simulink model "gtm_design"  (R2021b)
settings: Solver=ode15s  StartTime=0.0  StopTime=15  FixedStep=0.005  MaxStep=0.005  MinStep=0.0025
StopFcn:
  | MWSout=grabmws(bdroot);
  | MWSout.lastrun=datestr(now);
values from neighbouring files (symbols this model uses):
  s = tf('s')    [SingleDOF.m]    (also in main.m; newmain.m)
undefined symbols (not defined in the file or in its folder): Aero, aftfuel, aftfuel_pos, AILL, AILLC, AILR, AILRC, alpha_deg, altitude_ft, Ax_g, Ay_g, Az_g, b, beta_deg, bias, BRAKEC, Cbar, cg_pos0, cg_shift_gear, DamageCase, DamageModels, DamageOnsetTime, Earth, ELLIB, ELLIBC, ELLOB, ELLOBC, ELRIB, ELRIBC, ELROB, ELROBC, engl_ang, engl_pos, engr_ang, engr_pos, FLAPLIB, FLAPLIC, FLAPLOB, FLAPLOC, FLAPRIB, FLAPRIC, FLAPROB, FLAPROC, ft, FuelUsed_Init, fwdfuel, fwdfuel_pos, GEAR, GEARC, Inertia0, Inertia_shift_gear, Ixx_model, Iyy_model, Izz_model, KTAS, LandingGear, LengON, LinearizeModeOn, NAV_altitude_m, NAV_latitude_deg ... (+51)
libraries: simulink_extras x64, simulink_need_slupdate x30, LPVBlockLibrary x23, aerolibconvert2 x6, aerolibtransform2 x5, uavalgslib x4, UserContent_lib x3, simulink x3, robotcorelib x1, uavutilslib x1
(part 2 of 8)

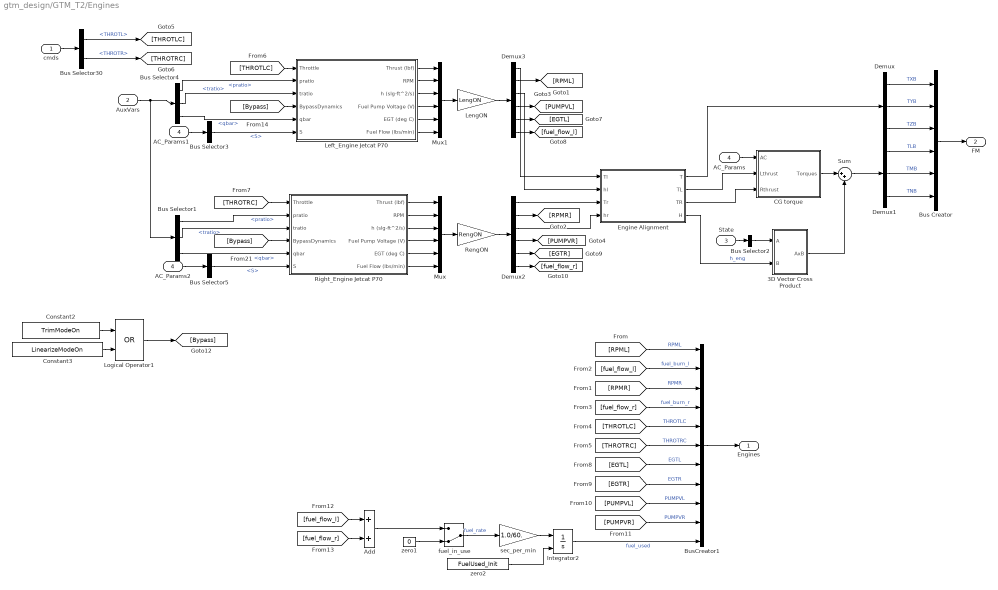
== system gtm_design/GTM_T2/Engines ==
  cmds : Inport
  AuxVars : Inport  Port=2
  State : Inport  Port=3
  AC_Params : Inport  Port=4
  3D Vector Cross Product : Subsystem
  AC_Params1 : InportShadow  Port=4
  AC_Params2 : InportShadow  Port=4
  Add : Sum
  Bus Creator : BusCreator  Inputs=6
  Bus Selector1 : BusSelector  OutputSignals=pratio,tratio,qbar
  Bus Selector2 : BusSelector  OutputSignals=pb,qb,rb  OutputAsBus=on
  Bus Selector3 : BusSelector  OutputSignals=S
  Bus Selector30 : BusSelector  OutputSignals=THROTL,THROTR
  Bus Selector4 : BusSelector  OutputSignals=pratio,tratio,qbar
  Bus Selector5 : BusSelector  OutputSignals=S
  BusCreator1 : BusCreator  Inputs=11
  CG torque : Subsystem
  Constant2 : Constant  Value=TrimModeOn
  Constant3 : Constant  Value=LinearizeModeOn
  Demux : Demux  Outputs=3
  Demux1 : Demux  Outputs=3
  Demux2 : Demux  Outputs=6
  Demux3 : Demux  Outputs=6
  Engine Alignment : MATLAB Function  TreatAsAtomicUnit=on
  Integrator2 : Integrator  InitialConditionSource=external
  Left_Engine Jetcat P70 : Subsystem
      mask init:
      | % Curve fit parameters for Jetcat P70 Model
      | % Coeff_thrust   = [0.000028864242464  -0.001914835880159 0.105916926095459  -1.251646340183624 ];
      | Coeff_thrust   = [0.000014847593013,  0, 0, 0.412662356277121];
      | Coeff_throttle = [0.000033035538475  -0.008354385314499 1.191126728328792 31.518959847101669];
      | Coeff_fuelflow = [0.000046800927870  -0.000779344124807 0.122178501497750];
      | Coeff_tau      = [ -2.2400e-02   2.9948e+00];
      | Coeff_EGT      = [ 2E-5, -0.0036,0.2342,-8.0496,664.99]; %EGT model, deg C
      | Coeff_dynamics = [ -.074 7.1];
      | fuelpump_table = [0 0.576	0.625	0.6985	0.7845	0.8575	0.919	0.9805	1.0415	1.1025...
      |                     1.1515	1.262	1.287	1.373	1.52	1.618	1.74	1.887	1.973...
      |                     2.12	2.255	2.4385	2.647	2.7575	2.9905	3.162]; %volts, table of fuel pump voltages
      | fuelflow_table = [0,0.0794,0.0876,0.102,0.1149,0.1275,0.1379,0.1487,0.1586,0.1671,...
      |                     0.1775,0.1858,0.194,0.2038,0.2206,0.2405,0.2566,0.2746,0.2921,0.3102,...
      |                     0.3266,0.3445,0.3533,0.3611,0.3866,0.4083;]*2; %lbs/min,   FULL fuel flow rates corresponding to pump voltages (fuelpump_table)  
      | % Equvalent Shaft parameters for engine
      | shaft_dia = 0.75/12.0;       % diameter of rotating turbine in feet 
      | shaft_len = 6.25/12.0;       % length of rotating turbine in feet   
      | density   = 15.2;            % mass density of steel in slugs/ft^3 
      | 
      | 
      | A = [-1.336,-0.7314;1,0;];
      | B = [1;0];
      | C = [-0.1474   0.7314];
      | D = 0;
  LengON : Gain  Gain=LengON  SaturateOnIntegerOverflow=on  OutDataTypeStr=Inherit: Same as input  ParamDataTypeStr=Inherit: Same as input
  Logical Operator1 : Logic  Operator=OR  AllPortsSameDT=off  OutDataTypeStr=boolean
  Mux : Mux  Inputs=6
  Mux1 : Mux  Inputs=6
  RengON : Gain  Gain=RengON  SaturateOnIntegerOverflow=on  OutDataTypeStr=Inherit: Same as input  ParamDataTypeStr=Inherit: Same as input
  Right_Engine Jetcat P70 : Subsystem
      mask init: same as gtm_design/GTM_T2/Engines/Left_Engine Jetcat P70
  Sum : Sum  Inputs=|++
  fuel_in_use : ManualSwitch  CurrentSetting=0
  sec_per_min : Gain  Gain=1.0/60.  SaturateOnIntegerOverflow=on  OutDataTypeStr=Inherit: Same as input  ParamDataTypeStr=Inherit: Same as input
  zero1 : Constant  Value=0
  zero2 : Constant  Value=FuelUsed_Init
  Engines : Outport
  FM : Outport  Port=2  PortDimensions=6
  wires:
  cmds/1 -> Bus Selector30/1
  Demux/2 -> Bus Creator/2  "TYB"
  State/1 -> Bus Selector2/1
  Bus Selector2/1 -> 3D Vector Cross Product/1(A)
  Demux/3 -> Bus Creator/3  "TZB"
  AuxVars/1 -> Bus Selector1/1, Bus Selector4/1
  AC_Params/1 -> CG torque/1(AC)
  Bus Creator/1 -> FM/1
  Bus Selector30/1 -> [THROTLC]  "<THROTL>"
  Bus Selector30/2 -> [THROTRC]  "<THROTR>"
  [THROTRC] -> BusCreator1/6  "THROTRC"
  [THROTLC] -> BusCreator1/5  "THROTLC"
  [fuel_flow_r] -> BusCreator1/4  "fuel_burn_r"
  [fuel_flow_l] -> BusCreator1/2  "fuel_burn_l"
  [RPMR] -> BusCreator1/3  "RPMR"
  [RPML] -> BusCreator1/1  "RPML"
  BusCreator1/1 -> Engines/1
  [EGTL] -> BusCreator1/7  "EGTL"
  [EGTR] -> BusCreator1/8  "EGTR"
  [PUMPVL] -> BusCreator1/9  "PUMPVL"
  [PUMPVR] -> BusCreator1/10  "PUMPVR"
  sec_per_min/1 -> Integrator2/1
  fuel_in_use/1 -> sec_per_min/1  "fuel_rate"
  Integrator2/1 -> BusCreator1/11  "fuel_used"
  zero2/1 -> Integrator2/2
  [fuel_flow_l] -> Add/1
  [fuel_flow_r] -> Add/2
  zero1/1 -> fuel_in_use/2
  Add/1 -> fuel_in_use/1
  Demux/1 -> Bus Creator/1  "TXB"
  Engine Alignment/4(H) -> 3D Vector Cross Product/2(B)  "h_eng"
  Engine Alignment/1(T) -> Demux/1
  Engine Alignment/2(TL) -> CG torque/2(Lthrust)
  Engine Alignment/3(TR) -> CG torque/3(Rthrust)
  CG torque/1(Torques) -> Sum/1
  3D Vector Cross Product/1(AxB) -> Sum/2
  Sum/1 -> Demux1/1
  Demux1/1 -> Bus Creator/4  "TLB"
  Demux1/2 -> Bus Creator/5  "TMB"
  Demux1/3 -> Bus Creator/6  "TNB"
  Mux/1 -> RengON/1
  RengON/1 -> Demux2/1
  Demux2/1 -> Engine Alignment/3(Tr)
  Demux2/2 -> [RPMR]
  Demux2/3 -> Engine Alignment/4(hr)
  Demux2/4 -> [PUMPVR]
  Demux2/5 -> [EGTR]
  Demux2/6 -> [fuel_flow_r]
  Mux1/1 -> LengON/1
  LengON/1 -> Demux3/1
  Demux3/1 -> Engine Alignment/1(Tl)
  Demux3/2 -> [RPML]
  Demux3/3 -> Engine Alignment/2(hl)
  Demux3/4 -> [PUMPVL]
  Demux3/5 -> [EGTL]
  Demux3/6 -> [fuel_flow_l]
  Constant3/1 -> Logical Operator1/2
  Constant2/1 -> Logical Operator1/1
  Logical Operator1/1 -> [Bypass]
  Left_Engine Jetcat P70/1(Thrust (lbf)) -> Mux1/1
  Left_Engine Jetcat P70/2(RPM) -> Mux1/2
  Left_Engine Jetcat P70/3(h (slg-ft^2/s)) -> Mux1/3
  Left_Engine Jetcat P70/4(Fuel Pump Voltage (V)) -> Mux1/4
  Left_Engine Jetcat P70/5(EGT (deg C)) -> Mux1/5
  Left_Engine Jetcat P70/6(Fuel Flow (lbs/min)) -> Mux1/6
  Right_Engine Jetcat P70/1(Thrust (lbf)) -> Mux/1
  Right_Engine Jetcat P70/2(RPM) -> Mux/2
  Right_Engine Jetcat P70/3(h (slg-ft^2/s)) -> Mux/3
  Right_Engine Jetcat P70/4(Fuel Pump Voltage (V)) -> Mux/4
  Right_Engine Jetcat P70/5(EGT (deg C)) -> Mux/5
  Right_Engine Jetcat P70/6(Fuel Flow (lbs/min)) -> Mux/6
  AC_Params2/1 -> Bus Selector5/1
  AC_Params1/1 -> Bus Selector3/1
  [THROTRC] -> Right_Engine Jetcat P70/1(Throttle)
  [THROTLC] -> Left_Engine Jetcat P70/1(Throttle)
  Bus Selector4/1 -> Left_Engine Jetcat P70/2(pratio)  "<pratio>"
  Bus Selector4/2 -> Left_Engine Jetcat P70/3(tratio)  "<tratio>"
  [Bypass] -> Left_Engine Jetcat P70/4(BypassDynamics)
  Bus Selector4/3 -> Left_Engine Jetcat P70/5(qbar)  "<qbar>"
  Bus Selector3/1 -> Left_Engine Jetcat P70/6(S)  "<S>"
  Bus Selector1/1 -> Right_Engine Jetcat P70/2(pratio)  "<pratio>"
  Bus Selector1/2 -> Right_Engine Jetcat P70/3(tratio)  "<tratio>"
  [Bypass] -> Right_Engine Jetcat P70/4(BypassDynamics)
  Bus Selector1/3 -> Right_Engine Jetcat P70/5(qbar)  "<qbar>"
  Bus Selector5/1 -> Right_Engine Jetcat P70/6(S)  "<S>"

== system gtm_design/GTM_T2/Gravity ==
  AuxVars : Inport
  Params : Inport  Port=2
  Bus Selector1 : BusSelector  OutputSignals=DCM
  Bus Selector6 : BusSelector  OutputSignals=mass
  Ground : Ground
  Ground1 : Ground
  Mux : Mux  Inputs=[3 3]
  Mux1 : Mux  Inputs=3
  Product : Product  Multiplication=Matrix(*)  RndMeth=Zero
  Product1 : Product  RndMeth=Zero
  acc due to gravity (ft/s^2) : Constant  Value=32.17405
  FM : Outport
  wires:
  acc due to gravity (ft/s^2)/1 -> Product1/2
  Ground1/1 -> Mux/2
  Product1/1 -> Mux1/3
  Ground/1 -> Mux1/2, Mux1/1
  Mux1/1 -> Product/2
  Mux/1 -> FM/1
  Product/1 -> Mux/1
  Params/1 -> Bus Selector6/1
  AuxVars/1 -> Bus Selector1/1
  Bus Selector1/1 -> Product/1  "<DCM>"
  Bus Selector6/1 -> Product1/1  "<mass>"

== system gtm_design/GTM_T2/Landing Gear ==
  State : Inport
  Surfaces : Inport  Port=2
  ACParams : Inport  Port=3
  Bus Selector : BusSelector  OutputSignals=BRAKE,STEER,GEAR
  Bus Selector1 : BusSelector  OutputSignals=pb,qb,rb  OutputAsBus=on
  Bus Selector2 : BusSelector  OutputSignals=ub,vb,wb  OutputAsBus=on
  Bus Selector3 : BusSelector  OutputSignals=psi
  Bus Selector4 : BusSelector  OutputSignals=altitude
  Bus Selector5 : BusSelector  OutputSignals=phi,theta,psi  OutputAsBus=on
  Bus Selector6 : BusSelector  OutputSignals=CG  OutputAsBus=on
  Bus to Vector : BusToVector
  Bus to Vector1 : BusToVector
  Bus to Vector2 : BusToVector
  Gain : Gain  Gain=1/100
  LandingGear : Subsystem  mask{NoseWheelPos=LandingGear.NoseWheelPos, LeftMainPos=LandingGear.LeftMainPos, RightMainPos=LandingGear.RightMainPos, SpringConst=LandingGear.SpringConst, DampingConst=LandingGear.DampingConst, StrokeLength=LandingGear.StrokeLength, MountStiffness=LandingGear.MountStiff, MountDamping=LandingGear.MountDamping, RunwayAlt=runway_alt}
      mask prompts: NoseWheelPos "Nose Wheel Position [X,Y,Z]"; LeftMainPos "Left Main Position [X,Y,Z]"; RightMainPos "Right Main Position [X,Y,Z]"; SpringConst "Spring Constant [Nose,Left,Right]"; DampingConst "Damping Constant [Nose,Left,Right]"; StrokeLength "Stroke Length [Nose,Left,Right]"; MountStiffness "Mount Stiffness [Nose,Left,Right]"; MountDamping "Mount Damping [Nose,Left, Right]"; RunwayAlt "Runway Altitude"
      mask help:
      | Implements ground reaction force (if geardown is nonzero) for 3-wheel landing gear. Linear stiffness and damping are applied within stroke range, and (generally larger) mount stiffness and damping are applied beyond this range.
      |
      | Underlying gear.c function is from HL-20/LaRCsim, e.b.jackson@nasa.gov
  Mux : Mux  Inputs=2
  FM : Outport
  GearState : Outport  Port=2
  wires:
  Mux/1 -> FM/1
  Gain/1 -> LandingGear/7(Brake (0-1))
  LandingGear/3(Contact) -> GearState/1
  LandingGear/2(M_gear) -> Mux/2
  LandingGear/1(F_gear) -> Mux/1
  Bus Selector/3 -> LandingGear/9(geardown (0/1))  "<GEAR>"
  Bus Selector/2 -> LandingGear/8(Steer (deg))  "<STEER>"
  Bus Selector/1 -> Gain/1  "<BRAKE>"
  Bus Selector3/1 -> LandingGear/6(Heading (Rad))  "<psi>"
  Bus to Vector/1 -> LandingGear/4(pqr (Rad/sec))
  Bus Selector4/1 -> LandingGear/3(Altitude (ft))  "<altitude>"
  Bus to Vector2/1 -> LandingGear/2(EulerAngles (Rad))
  Bus Selector6/1 -> LandingGear/1(cg)
  Surfaces/1 -> Bus Selector/1
  State/1 -> Bus Selector1/1, Bus Selector2/1, Bus Selector3/1, Bus Selector4/1, Bus Selector5/1
  Bus Selector1/1 -> Bus to Vector/1
  Bus to Vector1/1 -> LandingGear/5(Vbody (ft/sec))
  Bus Selector2/1 -> Bus to Vector1/1
  Bus Selector5/1 -> Bus to Vector2/1
  ACParams/1 -> Bus Selector6/1

== system gtm_design/GTM_T2/Sensors ==
  EOM_State : Inport
  EOM_Xdot : Inport  Port=2
  AC_Params : Inport  Port=3
  AuxVars : Inport  Port=4
  SurfacePos : Inport  Port=5
  Engines : Inport  Port=6
  Air Data : Subsystem
  AuxVars1 : InportShadow  Port=4
  Bus Creator : BusCreator  Inputs=5
  Engine ECU 8 Hz : Subsystem  SystemSampleTime=round(1/Timestep/8)*Timestep
  MAG3 IMU : Subsystem
  MIDG II 50 Hz : Subsystem  SystemSampleTime=round(1/Timestep/50)*Timestep
  Surface Pots : Subsystem
  Terminator : Terminator
  Terminator1 : Terminator
  Sensors : Outport
  wires:
  AC_Params/1 -> Terminator1/1
  EOM_Xdot/1 -> Terminator/1
  Bus Creator/1 -> Sensors/1
  Air Data/1(AirData) -> Bus Creator/1  "AirData"
  MIDG II 50 Hz/1(MIDG) -> Bus Creator/2  "MIDG"
  Surface Pots/1(Pots) -> Bus Creator/4  "SurfacePos"
  Engine ECU 8 Hz/1(ECU) -> Bus Creator/5  "Engines"
  MAG3 IMU/1(MAG3) -> Bus Creator/3  "MAG3"
  Engines/1 -> Engine ECU 8 Hz/1(Engines)
  SurfacePos/1 -> Surface Pots/1(SurfacePos)
  AuxVars/1 -> Air Data/2(AuxVars), MIDG II 50 Hz/1(AuxVars)
  EOM_State/1 -> MIDG II 50 Hz/2(EOM_State), Air Data/1(EOM_State), MAG3 IMU/2(EOM_State)
  AuxVars1/1 -> MAG3 IMU/1(AuxVars)

== system gtm_design/GTM_T2/TransportDelay ==
  note: Uplink Path
  note: Downlink Path
  Sensors : Inport
  UL : Inport  Port=2
  AntiAliasing : Subsystem
  Transport Delay on Bus : Subsystem
  Transport Delay on Bus1 : Subsystem
  cmds : Outport
  DL : Outport  Port=2
  wires:
  AntiAliasing/1(O) -> Transport Delay on Bus/1(In)
  Transport Delay on Bus/1(Out) -> DL/1
  UL/1 -> Transport Delay on Bus1/1(In)
  Sensors/1 -> AntiAliasing/1(I)
  Transport Delay on Bus1/1(Out) -> cmds/1

== system gtm_design/Navigation and Guidance/High-G Turn ==
  Add : Sum  Inputs=++++
  Add1 : Sum  Inputs=++++
  Constant{,1..2,4..6} (6 alike) : Constant  Value=0
  Constant3 : Constant  Value=-1
  Gain : Gain
  Gain1 : Gain
  Mux : Mux  Inputs=3
  Step : Step  After=80  SampleTime=0
  Step3 : Step  Time=10  After=5  SampleTime=0
  Out1 : Outport
  wires:
  Gain/1 -> Mux/3
  Step/1 -> Add/2  "1"
  Constant/1 -> Mux/2
  Mux/1 -> Out1/1
  Add1/1 -> Gain1/1
  Add/1 -> Gain/1
  Constant1/1 -> Add/1
  Constant3/1 -> Add1/1
  Step3/1 -> Add1/2  "1"
  Gain1/1 -> Mux/1
  Constant2/1 -> Add1/3
  Constant4/1 -> Add1/4
  Constant5/1 -> Add/3
  Constant6/1 -> Add/4

== system gtm_design/Navigation and Guidance/Lateral Doublet ==
  Add : Sum  Inputs=++++
  Constant1 : Constant  Value=0
  Constant2 : Constant  Value=-1
  Constant3 : Constant  Value=0
  Gain : Gain  Gain=3
  Gain1 : Gain  Gain=0
  Mux : Mux  Inputs=3
  Step : Step  SampleTime=0
  Step1 : Step  Time=5  After=-2  SampleTime=0
  Step2 : Step  Time=9  SampleTime=0
  Out1 : Outport
  wires:
  Mux/1 -> Out1/1
  Step2/1 -> Add/4  "1"
  Step1/1 -> Add/3  "-2"
  Step/1 -> Add/2  "1"
  Constant2/1 -> Mux/1
  Add/1 -> Gain1/1, Gain/1
  Constant1/1 -> Add/1
  Gain/1 -> Mux/3
  Gain1/1 -> Mux/2

== system gtm_design/Navigation and Guidance/Longitudinal Doublet ==
  Add : Sum  Inputs=++++
  Constant : Constant  Value=0
  Constant1 : Constant  Value=-1
  Constant2 : Constant  Value=0
  Gain : Gain
  Mux : Mux  Inputs=3
  Step : Step  SampleTime=0
  Step1 : Step  Time=3  After=-3  SampleTime=0
  Step2 : Step  Time=5  After=2  SampleTime=0
  Out1 : Outport
  wires:
  Mux/1 -> Out1/1
  Constant/1 -> Mux/2
  Step/1 -> Add/2
  Step1/1 -> Add/3
  Constant1/1 -> Add/1
  Step2/1 -> Add/4
  Add/1 -> Gain/1
  Constant2/1 -> Mux/3
  Gain/1 -> Mux/1

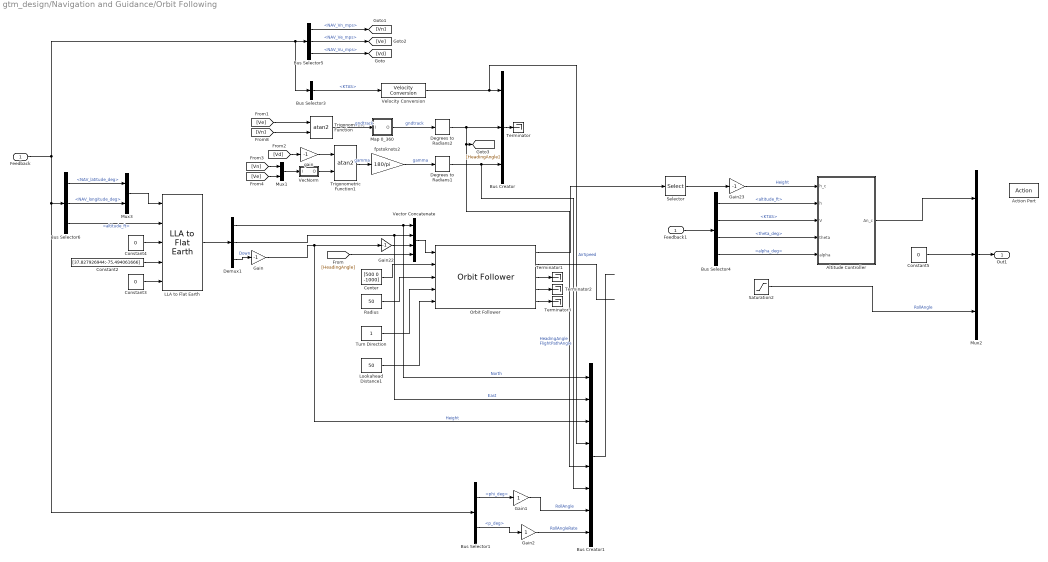
== system gtm_design/Navigation and Guidance/Orbit Following ==
  Feedback : Inport
  Action Port : ActionPort  ActionPortLabel=case [ 6 ]:
  Altitude Controller : MATLAB Function  TreatAsAtomicUnit=on
  Bus Creator : BusCreator  Inputs=3
  Bus Creator1 : BusCreator  Inputs=8
  Bus Selector1 : BusSelector  OutputSignals=MIDG.phi_deg,MAG3.p_deg
  Bus Selector3 : BusSelector  OutputSignals=AirData.KTAS
  Bus Selector4 : BusSelector  OutputSignals=AirData.altitude_ft,AirData.KTAS,MIDG.theta_deg,AirData.alpha_deg
  Bus Selector5 : BusSelector  OutputSignals=MIDG.NAV_Vn_mps,MIDG.NAV_Ve_mps,MIDG.NAV_Vu_mps
  Bus Selector6 : BusSelector  OutputSignals=MIDG.NAV_latitude_deg,MIDG.NAV_longitude_deg,AirData.altitude_ft
  Center : Constant  Value=[500 0 -1000]
  Constant2 : Constant  Value=[37.827926944;-75.494061666]
  Constant3 : Constant  Value=0
  Constant4 : Constant  Value=0
  Constant5 : Constant  Value=0
  Degrees to Radians1 : simulink_extras/Transformations/Degrees to Radians
  Degrees to Radians2 : simulink_extras/Transformations/Degrees to Radians
  Demux1 : Demux  Outputs=3
      settings: DisplayOption=none
  Feedback1 : InportShadow
  Gain : Gain  Gain=-1
  Gain1 : Gain
  Gain2 : Gain
  Gain22 : Gain  Gain=-1
  Gain23 : Gain  Gain=-1
  LLA to Flat Earth : aerolibtransform2/LLA to Flat Earth  units=English  ptype=Earth (WGS84)  F=1/298.257223563  R=20925646.3255  refPosPort=on  LL0=[0 10]  psi=0
      settings: SourceProductBaseCode=AE
  Lookahead Distance1 : Constant  Value=50
  Map 0_360 : Subsystem
  Mux1 : Mux  Inputs=2
  Mux2 : Mux  Inputs=3
  Mux3 : Mux  Inputs=2
  Orbit Follower : uavalgslib/Orbit Follower  UAVType=fixed-wing  MinOrbitRadius=1  MinLookaheadDistance=0.1  ExternalReset=none  ShowCrossTrackErrorOutput=off  ShowNumTurnsOutput=off  SimulateUsing=Interpreted execution
      settings: SourceProductBaseCode=UV
  Radius : Constant  Value=50
  Saturation2 : Saturate  UpperLimit=20/180*pi  LowerLimit=-20/180*pi
  Selector : Selector  InputPortWidth=3  IndexOptions=Index vector (dialog)  Indices=[3]  OutputSizes=1
  Terminator{,1..3} (4 alike) : Terminator
  Trigonometric Function : Trigonometry  Operator=atan2
  Trigonometric Function1 : Trigonometry  Operator=atan2
  Turn Direction : Constant
  VecNorm : Subsystem
  Vector Concatenate : Concatenate  NumInputs=4
  Velocity Conversion : aerolibconvert2/Velocity Conversion  IU=kts  OU=ft/s
  fpstoknots2 : Gain  Gain=180/pi
  gain : Gain  Gain=-1
  Out1 : Outport
  wires:
  Mux2/1 -> Out1/1
  Altitude Controller/1(An_c) -> Mux2/1
  [Vd] -> gain/1
  [Vn] -> Trigonometric Function/2
  fpstoknots2/1 -> Degrees to Radians1/1  "gamma"
  VecNorm/1(O) -> Trigonometric Function1/2
  Bus Selector5/2 -> [Ve]  "<NAV_Ve_mps>"
  Bus Selector3/1 -> Velocity Conversion/1  "<KTAS>"
  Bus Selector5/3 -> [Vd]  "<NAV_Vu_mps>"
  Feedback1/1 -> Bus Selector4/1
  Demux1/3 -> Gain/1  "Down"
  Bus Selector4/1 -> Altitude Controller/2(h)  "<altitude_ft>"
  Bus Selector6/2 -> Mux3/2  "<NAV_longitude_deg>"
  Bus Selector6/1 -> Mux3/1  "<NAV_latitude_deg>"
  Constant4/1 -> LLA to Flat Earth/3
  Orbit Follower/4 -> Terminator2/1
  [Ve] -> Trigonometric Function/1
  [Ve] -> Mux1/2
  [Vn] -> Mux1/1
  ? -> Saturation2/1
  Selector/1 -> Gain23/1
  Map 0_360/1(O) -> Degrees to Radians2/1  "gndtrack"
  [HeadingAngle] -> Vector Concatenate/4
  Bus Selector5/1 -> [Vn]  "<NAV_Vn_mps>"
  Orbit Follower/2 -> ?
  Constant3/1 -> LLA to Flat Earth/5
  Mux1/1 -> VecNorm/1(I)
  Gain22/1 -> Vector Concatenate/3
  Orbit Follower/3 -> Terminator1/1
  Orbit Follower/1 -> Selector/1
  Demux1/1 -> Bus Creator1/1, Vector Concatenate/1  "North"
  LLA to Flat Earth/1 -> Demux1/1
  gain/1 -> Trigonometric Function1/1
  Mux3/1 -> LLA to Flat Earth/1
  Bus Selector4/4 -> Altitude Controller/5(alpha)  "<alpha_deg>"
  Saturation2/1 -> Mux2/3  "RollAngle"
  Trigonometric Function/1 -> Map 0_360/1(I)  "gndtrack"
  Vector Concatenate/1 -> Orbit Follower/1
  Constant5/1 -> Mux2/2
  Bus Selector4/3 -> Altitude Controller/4(theta)  "<theta_deg>"
  Bus Selector4/2 -> Altitude Controller/3(V)  "<KTAS>"
  Trigonometric Function1/1 -> fpstoknots2/1  "gamma"
  Gain23/1 -> Altitude Controller/1(h_c)  "Height"
  Bus Selector6/3 -> LLA to Flat Earth/2  "<altitude_ft>"
  Constant2/1 -> LLA to Flat Earth/4
  Center/1 -> Orbit Follower/2
  Radius/1 -> Orbit Follower/3
  Turn Direction/1 -> Orbit Follower/4
  Lookahead Distance1/1 -> Orbit Follower/5
  Orbit Follower/5 -> Terminator3/1
  Gain/1 -> Bus Creator1/3, Gain22/1  "Height"
  Degrees to Radians2/1 -> Bus Creator/2, Bus Creator1/5, [HeadingAngle]  "HeadingAngle"
  Gain1/1 -> Bus Creator1/7  "RollAngle"
  Gain2/1 -> Bus Creator1/8  "RollAngleRate"
  Bus Creator1/1 -> ?
  Feedback/1 -> Bus Selector3/1, Bus Selector5/1, Bus Selector1/1, Bus Selector6/1
  Demux1/2 -> Bus Creator1/2, Vector Concatenate/2  "East"
  Bus Selector1/1 -> Gain1/1  "<phi_deg>"
  Bus Selector1/2 -> Gain2/1  "<p_deg>"
  Velocity Conversion/1 -> Bus Creator1/4, Bus Creator/1  "AirSpeed"
  Degrees to Radians1/1 -> Bus Creator1/6, Bus Creator/3  "FlightPathAngle"
  Bus Creator/1 -> Terminator/1

== system gtm_design/Navigation and Guidance/Pushover and Pullup ==
  Add : Sum  Inputs=++++
  Constant : Constant  Value=0
  Constant1 : Constant  Value=-1
  Constant2 : Constant  Value=0
  Constant3 : Constant  Value=0
  Gain : Gain
  Mux : Mux  Inputs=3
  Step : Step  SampleTime=0
  Step1 : Step  Time=15  After=4  SampleTime=0
  Out1 : Outport
  wires:
  Mux/1 -> Out1/1
  Constant2/1 -> Mux/3
  Add/1 -> Gain/1
  Constant1/1 -> Add/1
  Step1/1 -> Add/3
  Constant/1 -> Mux/2
  Step/1 -> Add/2
  Gain/1 -> Mux/1
  Constant3/1 -> Add/4

== system gtm_design/Navigation and Guidance/Straight and Level Flight ==
  Feedback1 : Inport
  Altitude Controller : MATLAB Function  TreatAsAtomicUnit=on
  Bus Selector3 : BusSelector  OutputSignals=AirData.altitude_ft,AirData.KTAS,MIDG.theta_deg,AirData.alpha_deg
  Constant : Constant  Value=0
  Constant2 : Constant  Value=0
  Constant3 : Constant  Value=1000
  Gain : Gain  Gain=1/32.17405
  Mux : Mux  Inputs=3
  Scope : Scope
  Out1 : Outport
  wires:
  Constant/1 -> Mux/2
  Mux/1 -> Out1/1
  Constant2/1 -> Mux/3
  Feedback1/1 -> Bus Selector3/1
  Bus Selector3/2 -> Altitude Controller/3(V)  "<KTAS>"
  Bus Selector3/3 -> Altitude Controller/4(theta)  "<theta_deg>"
  Bus Selector3/1 -> Scope/1, Altitude Controller/2(h)  "<altitude_ft>"
  Bus Selector3/4 -> Altitude Controller/5(alpha)  "<alpha_deg>"
  Constant3/1 -> Altitude Controller/1(h_c)
  Altitude Controller/1(Az_c) -> Gain/1
  Gain/1 -> Mux/1

== system gtm_design/Navigation and Guidance/Straight and Level Flight1 ==
  Constant : Constant  Value=0
  Constant1 : Constant
  Constant2 : Constant  Value=0
  Mux : Mux  Inputs=3
  Out1 : Outport
  wires:
  Constant1/1 -> Mux/1
  Constant2/1 -> Mux/3
  Mux/1 -> Out1/1
  Constant/1 -> Mux/2

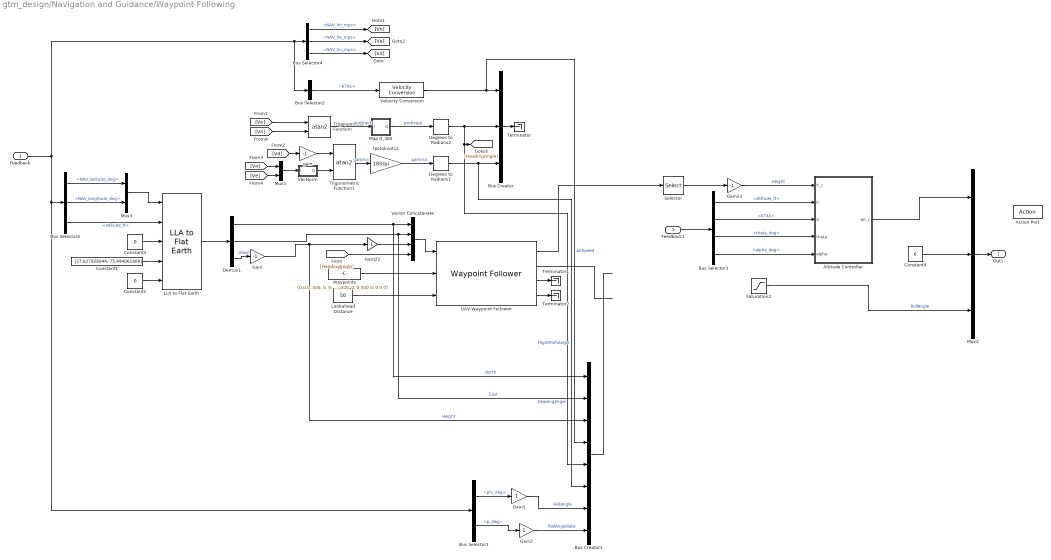
== system gtm_design/Navigation and Guidance/Waypoint Following ==
  Feedback : Inport
  Action Port : ActionPort  ActionPortLabel=case [ 5 ]:
  Altitude Controller : MATLAB Function  TreatAsAtomicUnit=on
  Bus Creator : BusCreator  Inputs=3
  Bus Creator1 : BusCreator  Inputs=8
  Bus Selector1 : BusSelector  OutputSignals=MIDG.phi_deg,MAG3.p_deg
  Bus Selector2 : BusSelector  OutputSignals=AirData.KTAS
  Bus Selector3 : BusSelector  OutputSignals=AirData.altitude_ft,AirData.KTAS,MIDG.theta_deg,AirData.alpha_deg
  Bus Selector4 : BusSelector  OutputSignals=MIDG.NAV_Vn_mps,MIDG.NAV_Ve_mps,MIDG.NAV_Vu_mps
  Bus Selector5 : BusSelector  OutputSignals=MIDG.NAV_latitude_deg,MIDG.NAV_longitude_deg,AirData.altitude_ft
  Constant1 : Constant  Value=[37.827926944;-75.494061666]
  Constant2 : Constant  Value=0
  Constant3 : Constant  Value=0
  Constant4 : Constant  Value=0
  Degrees to Radians1 : simulink_extras/Transformations/Degrees to Radians
  Degrees to Radians2 : simulink_extras/Transformations/Degrees to Radians
  Demux1 : Demux  Outputs=3
      settings: DisplayOption=none
  Feedback1 : InportShadow
  Gain : Gain  Gain=-1
  Gain1 : Gain
  Gain2 : Gain
  Gain22 : Gain  Gain=-1
  Gain23 : Gain  Gain=-1
  LLA to Flat Earth : aerolibtransform2/LLA to Flat Earth  units=English  ptype=Earth (WGS84)  F=1/298.257223563  R=20925646.3255  refPosPort=on  LL0=[0 10]  psi=0
      settings: SourceProductBaseCode=AE
  Lookahead Distance : Constant  Value=50
  Map 0_360 : Subsystem
  Mux1 : Mux  Inputs=2
  Mux2 : Mux  Inputs=3
  Mux3 : Mux  Inputs=2
  Saturation2 : Saturate  UpperLimit=20/180*pi  LowerLimit=-20/180*pi
  Selector : Selector  InputPortWidth=3  IndexOptions=Index vector (dialog)  Indices=[3]  OutputSizes=1
  Terminator : Terminator
  Terminator1 : Terminator
  Terminator2 : Terminator
  Trigonometric Function : Trigonometry  Operator=atan2
  Trigonometric Function1 : Trigonometry  Operator=atan2
  UAV Waypoint Follower : uavalgslib/Waypoint Follower  UAVType=fixed-wing  StartFrom=first  TransitionRadiusSource=internal  TransitionRadius=10  MinLookaheadDistance=0.1  YawInput=off  ShowCrossTrackErrorOutput=off  ShowStatusOutput=off  SimulateUsing=Code generation
      settings: SourceProductBaseCode=UV
  VecNorm : Subsystem
  Vector Concatenate : Concatenate  NumInputs=4
  Velocity Conversion : aerolibconvert2/Velocity Conversion  IU=kts  OU=ft/s
  Waypoints : Constant  Value=[0,0,0; 500, 0, 0; 500, 500, 0; 0 500 0; 0 0 0]  VectorParams1D=off
  fpstoknots2 : Gain  Gain=180/pi
  gain : Gain  Gain=-1
  Out1 : Outport
  wires:
  UAV Waypoint Follower/3 -> Terminator1/1
  UAV Waypoint Follower/2 -> ?
  Selector/1 -> Gain23/1
  Gain23/1 -> Altitude Controller/1(h_c)  "Height"
  UAV Waypoint Follower/1 -> Selector/1
  ? -> Saturation2/1
  UAV Waypoint Follower/4 -> Terminator2/1
  Saturation2/1 -> Mux2/3  "RollAngle"
  Lookahead Distance/1 -> UAV Waypoint Follower/3
  Vector Concatenate/1 -> UAV Waypoint Follower/1
  Waypoints/1 -> UAV Waypoint Follower/2
  Trigonometric Function/1 -> Map 0_360/1(I)  "gndtrack"
  Degrees to Radians1/1 -> Bus Creator1/6, Bus Creator/3  "FlightPathAngle"
  Bus Selector4/2 -> [Ve]  "<NAV_Ve_mps>"
  VecNorm/1(O) -> Trigonometric Function1/2
  gain/1 -> Trigonometric Function1/1
  Map 0_360/1(O) -> Degrees to Radians2/1  "gndtrack"
  Trigonometric Function1/1 -> fpstoknots2/1  "gamma"
  fpstoknots2/1 -> Degrees to Radians1/1  "gamma"
  Bus Selector4/3 -> [Vd]  "<NAV_Vu_mps>"
  [Ve] -> Mux1/2
  [Vn] -> Trigonometric Function/2
  Degrees to Radians2/1 -> Bus Creator1/5, [HeadingAngle], Bus Creator/2  "HeadingAngle"
  [Ve] -> Trigonometric Function/1
  [Vd] -> gain/1
  [Vn] -> Mux1/1
  Bus Selector4/1 -> [Vn]  "<NAV_Vn_mps>"
  Mux1/1 -> VecNorm/1(I)
  Bus Selector2/1 -> Velocity Conversion/1  "<KTAS>"
  Velocity Conversion/1 -> Bus Creator1/4, Bus Creator/1  "AirSpeed"
  Feedback1/1 -> Bus Selector3/1
  Bus Selector3/2 -> Altitude Controller/3(V)  "<KTAS>"
  Bus Selector3/1 -> Altitude Controller/2(h)  "<altitude_ft>"
  Bus Selector3/3 -> Altitude Controller/4(theta)  "<theta_deg>"
  Bus Selector3/4 -> Altitude Controller/5(alpha)  "<alpha_deg>"
  Feedback/1 -> Bus Selector2/1, Bus Selector4/1, Bus Selector1/1, Bus Selector5/1
  Bus Selector5/1 -> Mux3/1  "<NAV_latitude_deg>"
  Mux3/1 -> LLA to Flat Earth/1
  Constant1/1 -> LLA to Flat Earth/4
  Bus Selector5/2 -> Mux3/2  "<NAV_longitude_deg>"
  Constant3/1 -> LLA to Flat Earth/3
  Constant2/1 -> LLA to Flat Earth/5
  Bus Selector5/3 -> LLA to Flat Earth/2  "<altitude_ft>"
  LLA to Flat Earth/1 -> Demux1/1
  Mux2/1 -> Out1/1
  Altitude Controller/1(An_c) -> Mux2/1
  Constant4/1 -> Mux2/2
  Gain22/1 -> Vector Concatenate/3
  Gain/1 -> Bus Creator1/3, Gain22/1  "Height"
  Demux1/1 -> Vector Concatenate/1, Bus Creator1/1  "North"
  [HeadingAngle] -> Vector Concatenate/4
  Demux1/2 -> Vector Concatenate/2, Bus Creator1/2  "East"
  Demux1/3 -> Gain/1  "Down"
  Bus Selector1/2 -> Gain2/1  "<p_deg>"
  Bus Selector1/1 -> Gain1/1  "<phi_deg>"
  Gain1/1 -> Bus Creator1/7  "RollAngle"
  Gain2/1 -> Bus Creator1/8  "RollAngleRate"
  Bus Creator1/1 -> ?
  Bus Creator/1 -> Terminator/1

== system gtm_design/Navigation and Guidance1/High-G Turn ==
  Action Port : ActionPort
  Add : Sum  Inputs=++++
  Add1 : Sum  Inputs=++++
  Constant{,1..2,4..6} (6 alike) : Constant  Value=0
  Constant3 : Constant
  Gain : Gain
  Gain1 : Gain
  Mux : Mux  Inputs=3
  Step : Step  After=80  SampleTime=0
  Step3 : Step  Time=10  After=4  SampleTime=0
  Out1 : Outport
  wires:
  Gain/1 -> Mux/3
  Step/1 -> Add/2  "1"
  Constant/1 -> Mux/2
  Mux/1 -> Out1/1
  Add1/1 -> Gain1/1
  Add/1 -> Gain/1
  Constant1/1 -> Add/1
  Constant3/1 -> Add1/1
  Step3/1 -> Add1/2  "1"
  Gain1/1 -> Mux/1
  Constant2/1 -> Add1/3
  Constant4/1 -> Add1/4
  Constant5/1 -> Add/3
  Constant6/1 -> Add/4

== system gtm_design/Navigation and Guidance1/Lateral Doublet ==
  Action Port : ActionPort
  Add : Sum  Inputs=++++
  Constant : Constant  Value=0
  Constant1 : Constant  Value=0
  Constant2 : Constant
  Gain : Gain  Gain=45
  Mux : Mux  Inputs=3
  Step : Step  SampleTime=0
  Step1 : Step  Time=5  After=-2  SampleTime=0
  Step2 : Step  Time=9  SampleTime=0
  Out1 : Outport
  wires:
  Mux/1 -> Out1/1
  Step2/1 -> Add/4  "1"
  Step1/1 -> Add/3  "-2"
  Constant/1 -> Mux/2
  Step/1 -> Add/2  "1"
  Constant2/1 -> Mux/1
  Add/1 -> Gain/1
  Gain/1 -> Mux/3
  Constant1/1 -> Add/1

== system gtm_design/Navigation and Guidance1/Longitudinal Doublet ==
  Action Port : ActionPort
  Add : Sum  Inputs=++++
  Constant : Constant  Value=0
  Constant1 : Constant
  Constant2 : Constant  Value=0
  Gain : Gain
  Mux : Mux  Inputs=3
  Step : Step  SampleTime=0
  Step1 : Step  Time=5  After=-2  SampleTime=0
  Step2 : Step  Time=9  SampleTime=0
  Out1 : Outport
  wires:
  Mux/1 -> Out1/1
  Constant/1 -> Mux/2
  Step/1 -> Add/2
  Step1/1 -> Add/3
  Constant1/1 -> Add/1
  Step2/1 -> Add/4
  Add/1 -> Gain/1
  Constant2/1 -> Mux/3
  Gain/1 -> Mux/1

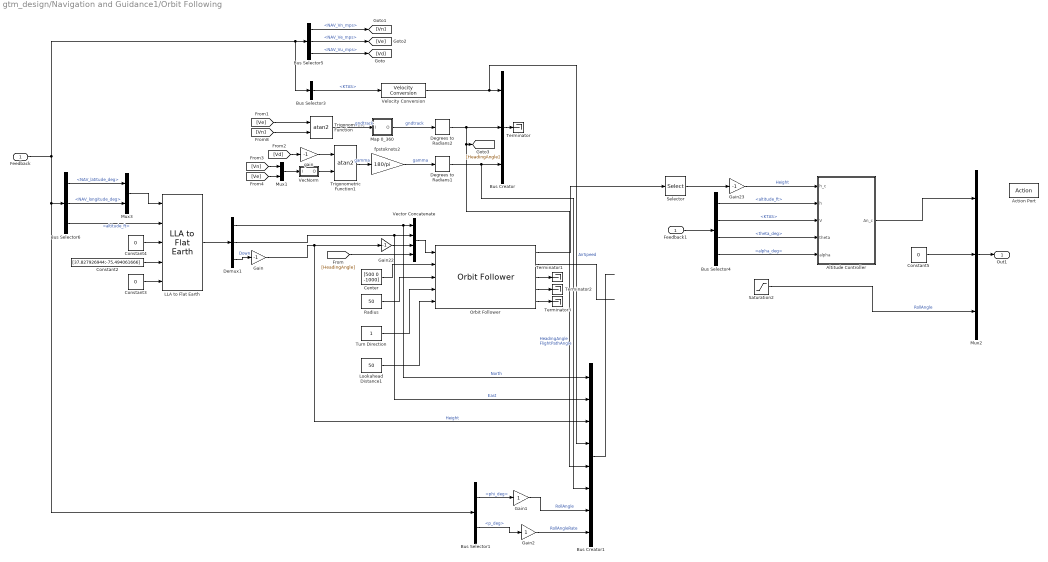
== system gtm_design/Navigation and Guidance1/Orbit Following ==
  Feedback : Inport
  Action Port : ActionPort
  Altitude Controller : MATLAB Function  TreatAsAtomicUnit=on
  Bus Creator : BusCreator  Inputs=3
  Bus Creator1 : BusCreator  Inputs=8
  Bus Selector1 : BusSelector  OutputSignals=MIDG.phi_deg,MAG3.p_deg
  Bus Selector3 : BusSelector  OutputSignals=AirData.KTAS
  Bus Selector4 : BusSelector  OutputSignals=AirData.altitude_ft,AirData.KTAS,MIDG.theta_deg,AirData.alpha_deg
  Bus Selector5 : BusSelector  OutputSignals=MIDG.NAV_Vn_mps,MIDG.NAV_Ve_mps,MIDG.NAV_Vu_mps
  Bus Selector6 : BusSelector  OutputSignals=MIDG.NAV_latitude_deg,MIDG.NAV_longitude_deg,AirData.altitude_ft
  Center : Constant  Value=[500 0 -1000]
  Constant2 : Constant  Value=[37.827926944;-75.494061666]
  Constant3 : Constant  Value=0
  Constant4 : Constant  Value=0
  Constant5 : Constant  Value=0
  Degrees to Radians1 : simulink_extras/Transformations/Degrees to Radians
  Degrees to Radians2 : simulink_extras/Transformations/Degrees to Radians
  Demux1 : Demux  Outputs=3
      settings: DisplayOption=none
  Feedback1 : InportShadow
  Gain : Gain  Gain=-1
  Gain1 : Gain
  Gain2 : Gain
  Gain22 : Gain  Gain=-1
  Gain23 : Gain  Gain=-1
  LLA to Flat Earth : aerolibtransform2/LLA to Flat Earth  units=English  ptype=Earth (WGS84)  F=1/298.257223563  R=20925646.3255  refPosPort=on  LL0=[0 10]  psi=0
      settings: SourceProductBaseCode=AE
  Lookahead Distance1 : Constant  Value=50
  Map 0_360 : Subsystem
  Mux1 : Mux  Inputs=2
  Mux2 : Mux  Inputs=3
  Mux3 : Mux  Inputs=2
  Orbit Follower : uavalgslib/Orbit Follower  UAVType=fixed-wing  MinOrbitRadius=1  MinLookaheadDistance=0.1  ExternalReset=none  ShowCrossTrackErrorOutput=off  ShowNumTurnsOutput=off  SimulateUsing=Interpreted execution
      settings: SourceProductBaseCode=UV
  Radius : Constant  Value=50
  Saturation2 : Saturate  UpperLimit=20/180*pi  LowerLimit=-20/180*pi
  Selector : Selector  InputPortWidth=3  IndexOptions=Index vector (dialog)  Indices=[3]  OutputSizes=1
  Terminator{,1..3} (4 alike) : Terminator
  Trigonometric Function : Trigonometry  Operator=atan2
  Trigonometric Function1 : Trigonometry  Operator=atan2
  Turn Direction : Constant
  VecNorm : Subsystem
  Vector Concatenate : Concatenate  NumInputs=4
  Velocity Conversion : aerolibconvert2/Velocity Conversion  IU=kts  OU=ft/s
  fpstoknots2 : Gain  Gain=180/pi
  gain : Gain  Gain=-1
  Out1 : Outport
  wires:
  Mux2/1 -> Out1/1
  Altitude Controller/1(An_c) -> Mux2/1
  [Vd] -> gain/1
  [Vn] -> Trigonometric Function/2
  fpstoknots2/1 -> Degrees to Radians1/1  "gamma"
  VecNorm/1(O) -> Trigonometric Function1/2
  Bus Selector5/2 -> [Ve]  "<NAV_Ve_mps>"
  Bus Selector3/1 -> Velocity Conversion/1  "<KTAS>"
  Bus Selector5/3 -> [Vd]  "<NAV_Vu_mps>"
  Feedback1/1 -> Bus Selector4/1
  Demux1/3 -> Gain/1  "Down"
  Bus Selector4/1 -> Altitude Controller/2(h)  "<altitude_ft>"
  Bus Selector6/2 -> Mux3/2  "<NAV_longitude_deg>"
  Bus Selector6/1 -> Mux3/1  "<NAV_latitude_deg>"
  Constant4/1 -> LLA to Flat Earth/3
  Orbit Follower/4 -> Terminator2/1
  [Ve] -> Trigonometric Function/1
  [Ve] -> Mux1/2
  [Vn] -> Mux1/1
  ? -> Saturation2/1
  Selector/1 -> Gain23/1
  Map 0_360/1(O) -> Degrees to Radians2/1  "gndtrack"
  [HeadingAngle] -> Vector Concatenate/4
  Bus Selector5/1 -> [Vn]  "<NAV_Vn_mps>"
  Orbit Follower/2 -> ?
  Constant3/1 -> LLA to Flat Earth/5
  Mux1/1 -> VecNorm/1(I)
  Gain22/1 -> Vector Concatenate/3
  Orbit Follower/3 -> Terminator1/1
  Orbit Follower/1 -> Selector/1
  Demux1/1 -> Bus Creator1/1, Vector Concatenate/1  "North"
  LLA to Flat Earth/1 -> Demux1/1
  gain/1 -> Trigonometric Function1/1
  Mux3/1 -> LLA to Flat Earth/1
  Bus Selector4/4 -> Altitude Controller/5(alpha)  "<alpha_deg>"
  Saturation2/1 -> Mux2/3  "RollAngle"
  Trigonometric Function/1 -> Map 0_360/1(I)  "gndtrack"
  Vector Concatenate/1 -> Orbit Follower/1
  Constant5/1 -> Mux2/2
  Bus Selector4/3 -> Altitude Controller/4(theta)  "<theta_deg>"
  Bus Selector4/2 -> Altitude Controller/3(V)  "<KTAS>"
  Trigonometric Function1/1 -> fpstoknots2/1  "gamma"
  Gain23/1 -> Altitude Controller/1(h_c)  "Height"
  Bus Selector6/3 -> LLA to Flat Earth/2  "<altitude_ft>"
  Constant2/1 -> LLA to Flat Earth/4
  Center/1 -> Orbit Follower/2
  Radius/1 -> Orbit Follower/3
  Turn Direction/1 -> Orbit Follower/4
  Lookahead Distance1/1 -> Orbit Follower/5
  Orbit Follower/5 -> Terminator3/1
  Gain/1 -> Bus Creator1/3, Gain22/1  "Height"
  Degrees to Radians2/1 -> Bus Creator/2, Bus Creator1/5, [HeadingAngle]  "HeadingAngle"
  Gain1/1 -> Bus Creator1/7  "RollAngle"
  Gain2/1 -> Bus Creator1/8  "RollAngleRate"
  Bus Creator1/1 -> ?
  Feedback/1 -> Bus Selector3/1, Bus Selector5/1, Bus Selector1/1, Bus Selector6/1
  Demux1/2 -> Bus Creator1/2, Vector Concatenate/2  "East"
  Bus Selector1/1 -> Gain1/1  "<phi_deg>"
  Bus Selector1/2 -> Gain2/1  "<p_deg>"
  Velocity Conversion/1 -> Bus Creator1/4, Bus Creator/1  "AirSpeed"
  Degrees to Radians1/1 -> Bus Creator1/6, Bus Creator/3  "FlightPathAngle"
  Bus Creator/1 -> Terminator/1

== system gtm_design/Navigation and Guidance1/Pushover and Pullup ==
  Action Port : ActionPort
  Add : Sum  Inputs=++++
  Constant : Constant  Value=0
  Constant1 : Constant
  Constant2 : Constant  Value=0
  Constant3 : Constant  Value=0
  Gain : Gain
  Mux : Mux  Inputs=3
  Step : Step  After=-1  SampleTime=0
  Step1 : Step  Time=15  After=4  SampleTime=0
  Out1 : Outport
  wires:
  Mux/1 -> Out1/1
  Constant2/1 -> Mux/3
  Add/1 -> Gain/1
  Constant1/1 -> Add/1
  Step1/1 -> Add/3
  Constant/1 -> Mux/2
  Step/1 -> Add/2
  Gain/1 -> Mux/1
  Constant3/1 -> Add/4

== system gtm_design/Navigation and Guidance1/Straight and Level Flight ==
  Action Port : ActionPort
  Constant : Constant  Value=0
  Constant1 : Constant
  Constant2 : Constant  Value=0
  Mux : Mux  Inputs=3
  Out1 : Outport
  wires:
  Constant/1 -> Mux/2
  Constant1/1 -> Mux/1
  Mux/1 -> Out1/1
  Constant2/1 -> Mux/3

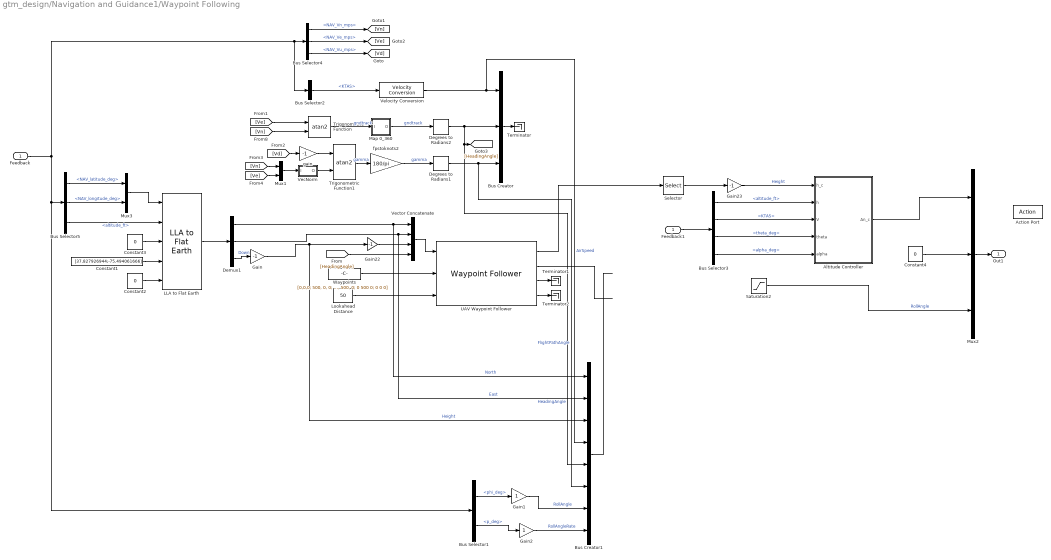
== system gtm_design/Navigation and Guidance1/Waypoint Following ==
  Feedback : Inport
  Action Port : ActionPort
  Altitude Controller : MATLAB Function  TreatAsAtomicUnit=on
  Bus Creator : BusCreator  Inputs=3
  Bus Creator1 : BusCreator  Inputs=8
  Bus Selector1 : BusSelector  OutputSignals=MIDG.phi_deg,MAG3.p_deg
  Bus Selector2 : BusSelector  OutputSignals=AirData.KTAS
  Bus Selector3 : BusSelector  OutputSignals=AirData.altitude_ft,AirData.KTAS,MIDG.theta_deg,AirData.alpha_deg
  Bus Selector4 : BusSelector  OutputSignals=MIDG.NAV_Vn_mps,MIDG.NAV_Ve_mps,MIDG.NAV_Vu_mps
  Bus Selector5 : BusSelector  OutputSignals=MIDG.NAV_latitude_deg,MIDG.NAV_longitude_deg,AirData.altitude_ft
  Constant1 : Constant  Value=[37.827926944;-75.494061666]
  Constant2 : Constant  Value=0
  Constant3 : Constant  Value=0
  Constant4 : Constant  Value=0
  Degrees to Radians1 : simulink_extras/Transformations/Degrees to Radians
  Degrees to Radians2 : simulink_extras/Transformations/Degrees to Radians
  Demux1 : Demux  Outputs=3
      settings: DisplayOption=none
  Feedback1 : InportShadow
  Gain : Gain  Gain=-1
  Gain1 : Gain
  Gain2 : Gain
  Gain22 : Gain  Gain=-1
  Gain23 : Gain  Gain=-1
  LLA to Flat Earth : aerolibtransform2/LLA to Flat Earth  units=English  ptype=Earth (WGS84)  F=1/298.257223563  R=20925646.3255  refPosPort=on  LL0=[0 10]  psi=0
      settings: SourceProductBaseCode=AE
  Lookahead Distance : Constant  Value=50
  Map 0_360 : Subsystem
  Mux1 : Mux  Inputs=2
  Mux2 : Mux  Inputs=3
  Mux3 : Mux  Inputs=2
  Saturation2 : Saturate  UpperLimit=20/180*pi  LowerLimit=-20/180*pi
  Selector : Selector  InputPortWidth=3  IndexOptions=Index vector (dialog)  Indices=[3]  OutputSizes=1
  Terminator : Terminator
  Terminator1 : Terminator
  Terminator2 : Terminator
  Trigonometric Function : Trigonometry  Operator=atan2
  Trigonometric Function1 : Trigonometry  Operator=atan2
  UAV Waypoint Follower : uavalgslib/Waypoint Follower  UAVType=fixed-wing  StartFrom=first  TransitionRadiusSource=internal  TransitionRadius=10  MinLookaheadDistance=0.1  YawInput=off  ShowCrossTrackErrorOutput=off  ShowStatusOutput=off  SimulateUsing=Code generation
      settings: SourceProductBaseCode=UV
  VecNorm : Subsystem
  Vector Concatenate : Concatenate  NumInputs=4
  Velocity Conversion : aerolibconvert2/Velocity Conversion  IU=kts  OU=ft/s
  Waypoints : Constant  Value=[0,0,0; 500, 0, 0; 500, 500, 0; 0 500 0; 0 0 0]  VectorParams1D=off
  fpstoknots2 : Gain  Gain=180/pi
  gain : Gain  Gain=-1
  Out1 : Outport
  wires:
  UAV Waypoint Follower/3 -> Terminator1/1
  UAV Waypoint Follower/2 -> ?
  Selector/1 -> Gain23/1
  Gain23/1 -> Altitude Controller/1(h_c)  "Height"
  UAV Waypoint Follower/1 -> Selector/1
  ? -> Saturation2/1
  UAV Waypoint Follower/4 -> Terminator2/1
  Saturation2/1 -> Mux2/3  "RollAngle"
  Lookahead Distance/1 -> UAV Waypoint Follower/3
  Vector Concatenate/1 -> UAV Waypoint Follower/1
  Waypoints/1 -> UAV Waypoint Follower/2
  Trigonometric Function/1 -> Map 0_360/1(I)  "gndtrack"
  Degrees to Radians1/1 -> Bus Creator1/6, Bus Creator/3  "FlightPathAngle"
  Bus Selector4/2 -> [Ve]  "<NAV_Ve_mps>"
  VecNorm/1(O) -> Trigonometric Function1/2
  gain/1 -> Trigonometric Function1/1
  Map 0_360/1(O) -> Degrees to Radians2/1  "gndtrack"
  Trigonometric Function1/1 -> fpstoknots2/1  "gamma"
  fpstoknots2/1 -> Degrees to Radians1/1  "gamma"
  Bus Selector4/3 -> [Vd]  "<NAV_Vu_mps>"
  [Ve] -> Mux1/2
  [Vn] -> Trigonometric Function/2
  Degrees to Radians2/1 -> Bus Creator1/5, [HeadingAngle], Bus Creator/2  "HeadingAngle"
  [Ve] -> Trigonometric Function/1
  [Vd] -> gain/1
  [Vn] -> Mux1/1
  Bus Selector4/1 -> [Vn]  "<NAV_Vn_mps>"
  Mux1/1 -> VecNorm/1(I)
  Bus Selector2/1 -> Velocity Conversion/1  "<KTAS>"
  Velocity Conversion/1 -> Bus Creator1/4, Bus Creator/1  "AirSpeed"
  Feedback1/1 -> Bus Selector3/1
  Bus Selector3/2 -> Altitude Controller/3(V)  "<KTAS>"
  Bus Selector3/1 -> Altitude Controller/2(h)  "<altitude_ft>"
  Bus Selector3/3 -> Altitude Controller/4(theta)  "<theta_deg>"
  Bus Selector3/4 -> Altitude Controller/5(alpha)  "<alpha_deg>"
  Feedback/1 -> Bus Selector2/1, Bus Selector4/1, Bus Selector1/1, Bus Selector5/1
  Bus Selector5/1 -> Mux3/1  "<NAV_latitude_deg>"
  Mux3/1 -> LLA to Flat Earth/1
  Constant1/1 -> LLA to Flat Earth/4
  Bus Selector5/2 -> Mux3/2  "<NAV_longitude_deg>"
  Constant3/1 -> LLA to Flat Earth/3
  Constant2/1 -> LLA to Flat Earth/5
  Bus Selector5/3 -> LLA to Flat Earth/2  "<altitude_ft>"
  LLA to Flat Earth/1 -> Demux1/1
  Mux2/1 -> Out1/1
  Altitude Controller/1(An_c) -> Mux2/1
  Constant4/1 -> Mux2/2
  Gain22/1 -> Vector Concatenate/3
  Gain/1 -> Bus Creator1/3, Gain22/1  "Height"
  Demux1/1 -> Vector Concatenate/1, Bus Creator1/1  "North"
  [HeadingAngle] -> Vector Concatenate/4
  Demux1/2 -> Vector Concatenate/2, Bus Creator1/2  "East"
  Demux1/3 -> Gain/1  "Down"
  Bus Selector1/2 -> Gain2/1  "<p_deg>"
  Bus Selector1/1 -> Gain1/1  "<phi_deg>"
  Gain1/1 -> Bus Creator1/7  "RollAngle"
  Gain2/1 -> Bus Creator1/8  "RollAngleRate"
  Bus Creator1/1 -> ?
  Bus Creator/1 -> Terminator/1

== system gtm_design/Subsystem2/Hinf ==
  Guidance : Inport
  Feedback : Inport  Port=2
  Add : Sum
  Bus Selector : BusSelector  OutputSignals=AirData.KTAS,AirData.altitude_ft,SurfacePos.AILL,SurfacePos.AILR
  Bus Selector3 : BusSelector  OutputSignals=An_c
  Bus Selector4 : BusSelector  OutputSignals=beta_c,phi_c  OutputAsBus=on
  Bus Selector5 : BusSelector  OutputSignals=AirData.alpha_deg,MAG3.q_deg,MAG3.Az_g
  Bus Selector6 : BusSelector  OutputSignals=AirData.beta_deg,MAG3.p_deg,MAG3.r_deg,MIDG.phi_deg,MAG3.Ay_g
  Bus to Vector : BusToVector
  Bus to Vector1 : BusToVector
  Constant : Constant
  Degrees to Radians{,1..5} (6 alike) : simulink_extras/Transformations/Degrees to Radians
  Demux1 : Demux  Outputs=2
  Gain : Gain  Gain=1/2
  Gain1 : Gain  Gain=1/100
  Gain2 : Gain  Gain=32.17405
  Gain3 : Gain  Gain=32.17405
  Gain4 : Gain  Gain=100
  Gain5 : Gain  Gain=100
  LPVBlock1 : LPVBlockLibrary/LPVBlock  sys=K_lon_hinf  plist={'rho1_tas_param';'rho2_alt_param';'rho3_mor_param'}  x0=0
      settings: SourceProductName=LPVTools Blocks
  LPVBlock2 : LPVBlockLibrary/LPVBlock  sys=K_lat_hinf  plist={'rho1_tas_param';'rho2_alt_param';'rho3_mor_param'}  x0=0
      settings: SourceProductName=LPVTools Blocks
  LPVBlock3 : LPVBlockLibrary/LPVBlock  sys=sch_alp_trim  plist={'rho1_tas_param';'rho2_alt_param';'rho3_mor_param'}  x0=0
      settings: SourceProductName=LPVTools Blocks
  Mux : Mux  Inputs=3
  Mux5 : Mux  Inputs=[1 1 1 1]
  Mux6 : Mux  Inputs=5
  Mux7 : Mux  Inputs=2
  Mux8 : Mux
  Radians to Degrees : simulink_extras/Transformations/Radians to Degrees
  Radians to Degrees1 : simulink_extras/Transformations/Radians to Degrees
  Selector : Selector  InputPortWidth=3  IndexOptions=Index vector (dialog)  Indices=3  OutputSizes=1
  Sum : Sum  Inputs=|+-
  Sum1 : Sum  Inputs=++|
  Sum2 : Sum  Inputs=|+-
  Out : Outport  InitialOutput=zeros(4,1)
  wires:
  Bus to Vector/1 -> Mux7/1
  Bus Selector4/1 -> Bus to Vector/1
  Bus to Vector1/1 -> Mux5/1
  Bus Selector3/1 -> Bus to Vector1/1  "<An_c>"
  Mux5/1 -> LPVBlock1/1
  Degrees to Radians/1 -> Mux5/2
  Degrees to Radians1/1 -> Mux5/3
  Gain2/1 -> Mux5/4
  Mux8/1 -> Out/1
  Radians to Degrees1/1 -> Mux8/1
  Gain4/1 -> Mux8/2
  Gain5/1 -> Mux8/3
  Radians to Degrees/1 -> Mux8/4
  Demux1/2 -> Radians to Degrees/1
  Sum1/1 -> Gain5/1
  Sum2/1 -> Gain4/1
  Demux1/1 -> Sum2/1, Sum1/2
  Selector/1 -> Sum2/2, Sum1/1
  [rho] -> Selector/1
  LPVBlock1/1 -> Radians to Degrees1/1
  LPVBlock2/1 -> Demux1/1
  [rho] -> LPVBlock2/2
  Mux7/1 -> LPVBlock2/1
  Mux6/1 -> Mux7/2
  Degrees to Radians5/1 -> Mux6/4
  Degrees to Radians4/1 -> Mux6/3
  Degrees to Radians3/1 -> Mux6/2
  Degrees to Radians2/1 -> Mux6/1
  Gain3/1 -> Mux6/5
  Bus Selector6/5 -> Gain3/1  "<Ay_g>"
  Bus Selector6/4 -> Degrees to Radians5/1  "<phi_deg>"
  Bus Selector6/3 -> Degrees to Radians4/1  "<r_deg>"
  Bus Selector6/2 -> Degrees to Radians3/1  "<p_deg>"
  Bus Selector6/1 -> Degrees to Radians2/1  "<beta_deg>"
  Sum/1 -> Degrees to Radians/1
  LPVBlock3/1 -> Sum/2
  Bus Selector5/2 -> Degrees to Radians1/1  "<q_deg>"
  [rho] -> LPVBlock3/2
  Constant/1 -> LPVBlock3/1
  [rho] -> LPVBlock1/2
  Bus Selector5/3 -> Gain2/1  "<Az_g>"
  Bus Selector5/1 -> Sum/1  "<alpha_deg>"
  Guidance/1 -> Bus Selector3/1, Bus Selector4/1
  Gain1/1 -> Mux/3
  Add/1 -> Gain/1
  Feedback/1 -> Bus Selector5/1, Bus Selector6/1, Bus Selector/1
  Bus Selector/1 -> Mux/1  "<KTAS>"
  Bus Selector/3 -> Add/1  "<AILL>"
  Bus Selector/4 -> Add/2  "<AILR>"
  Bus Selector/2 -> Mux/2  "<altitude_ft>"
  Gain/1 -> Gain1/1
  Mux/1 -> [rho]

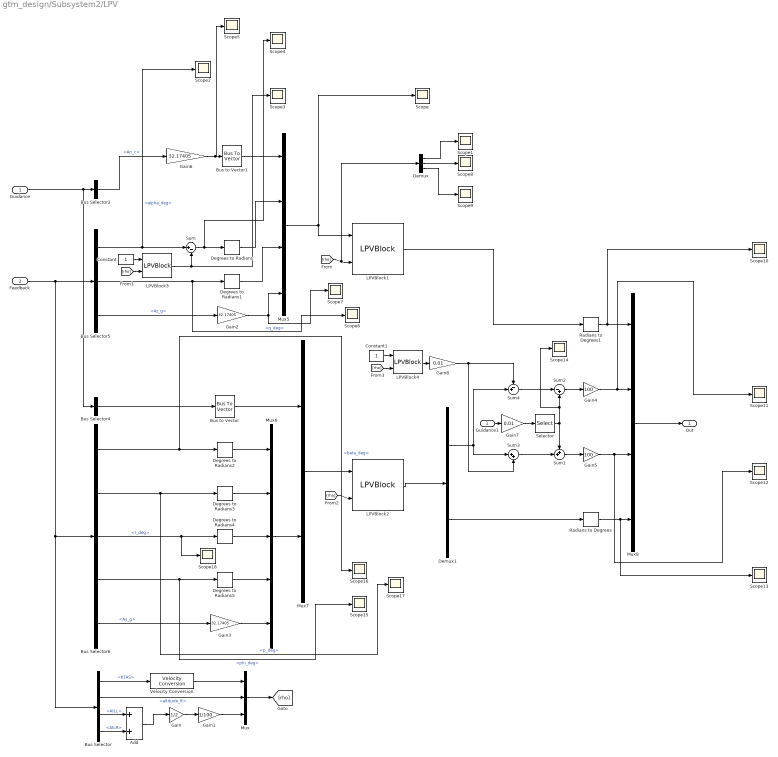
== system gtm_design/Subsystem2/LPV ==
  Guidance : Inport
  Feedback : Inport  Port=2
  Add : Sum
  Bus Selector : BusSelector  OutputSignals=AirData.KTAS,AirData.altitude_ft,SurfacePos.AILL,SurfacePos.AILR
  Bus Selector3 : BusSelector  OutputSignals=An_c
  Bus Selector4 : BusSelector  OutputSignals=beta_c,phi_c  OutputAsBus=on
  Bus Selector5 : BusSelector  OutputSignals=AirData.alpha_deg,MAG3.q_deg,MAG3.Az_g
  Bus Selector6 : BusSelector  OutputSignals=AirData.beta_deg,MAG3.p_deg,MAG3.r_deg,MIDG.phi_deg,MAG3.Ay_g
  Bus to Vector : BusToVector
  Bus to Vector1 : BusToVector
  Constant : Constant
  Constant1 : Constant
  Degrees to Radians{,1..5} (6 alike) : simulink_extras/Transformations/Degrees to Radians
  Demux : Demux  Outputs=3
  Demux1 : Demux  Outputs=2
  Gain : Gain  Gain=1/2
  Gain1 : Gain  Gain=1/100
  Gain2 : Gain  Gain=32.17405
  Gain3 : Gain  Gain=32.17405
  Gain4 : Gain  Gain=100
  Gain5 : Gain  Gain=100
  Gain6 : Gain  Gain=32.17405
  Gain7 : Gain  Gain=0.01
  Gain8 : Gain  Gain=0.01
  Guidance1 : InportShadow
  LPVBlock1 : LPVBlockLibrary/LPVBlock  sys=K_lon_lpv  plist={'rho1_tas_param';'rho2_alt_param';'rho3_mor_param'}  x0=0
      settings: SourceProductName=LPVTools Blocks
  LPVBlock2 : LPVBlockLibrary/LPVBlock  sys=K_lat_lpv  plist={'rho1_tas_param';'rho2_alt_param';'rho3_mor_param'}  x0=0
      settings: SourceProductName=LPVTools Blocks
  LPVBlock3 : LPVBlockLibrary/LPVBlock  sys=sch_alp_trim  plist={'rho1_tas_param';'rho2_alt_param';'rho3_mor_param'}  x0=0
      settings: SourceProductName=LPVTools Blocks
  LPVBlock4 : LPVBlockLibrary/LPVBlock  sys=sch_aileron_trim  plist={'rho1_tas_param';'rho2_alt_param';'rho3_mor_param'}  x0=0
      settings: SourceProductName=LPVTools Blocks
  Mux : Mux  Inputs=3
  Mux5 : Mux  Inputs=[1 1 1 1]
  Mux6 : Mux  Inputs=5
  Mux7 : Mux  Inputs=2
  Mux8 : Mux
  Radians to Degrees : simulink_extras/Transformations/Radians to Degrees
  Radians to Degrees1 : simulink_extras/Transformations/Radians to Degrees
  Scope{,1..18} (19 alike) : Scope
  Selector : Selector  InputPortWidth=5  IndexOptions=Index vector (dialog)  Indices=5  OutputSizes=1
  Sum : Sum  Inputs=|+-
  Sum1 : Sum  Inputs=++|
  Sum2 : Sum  Inputs=|-+
  Sum3 : Sum  Inputs=|++
  Sum4 : Sum  Inputs=-+|
  Velocity Conversion : aerolibconvert2/Velocity Conversion  IU=kts  OU=ft/s
  Out : Outport  InitialOutput=zeros(4,1)
  wires:
  Mux/1 -> [rho]
  Gain/1 -> Gain1/1
  Bus Selector/2 -> Mux/2  "<altitude_ft>"
  Bus Selector/4 -> Add/2  "<AILR>"
  Bus Selector/3 -> Add/1  "<AILL>"
  Bus Selector/1 -> Velocity Conversion/1  "<KTAS>"
  Feedback/1 -> Bus Selector/1, Bus Selector6/1, Bus Selector5/1
  Add/1 -> Gain/1
  Gain1/1 -> Mux/3
  Guidance/1 -> Bus Selector4/1, Bus Selector3/1
  Bus Selector5/1 -> Scope2/1, Sum/1  "<alpha_deg>"
  Bus Selector5/3 -> Gain2/1  "<Az_g>"
  [rho] -> Demux/1, LPVBlock1/2
  Constant/1 -> LPVBlock3/1
  [rho] -> LPVBlock3/2
  Bus Selector5/2 -> Scope6/1, Degrees to Radians1/1  "<q_deg>"
  LPVBlock3/1 -> Scope3/1, Sum/2
  Sum/1 -> Scope4/1, Degrees to Radians/1
  Bus Selector6/1 -> Scope16/1, Degrees to Radians2/1  "<beta_deg>"
  Bus Selector6/2 -> Scope17/1, Degrees to Radians3/1  "<p_deg>"
  Bus Selector6/3 -> Scope18/1, Degrees to Radians4/1  "<r_deg>"
  Bus Selector6/4 -> Scope15/1, Degrees to Radians5/1  "<phi_deg>"
  Bus Selector6/5 -> Gain3/1  "<Ay_g>"
  Gain3/1 -> Mux6/5
  Degrees to Radians2/1 -> Mux6/1
  Degrees to Radians3/1 -> Mux6/2
  Degrees to Radians4/1 -> Mux6/3
  Degrees to Radians5/1 -> Mux6/4
  Mux6/1 -> Mux7/2
  Mux7/1 -> LPVBlock2/1
  [rho] -> LPVBlock2/2
  LPVBlock2/1 -> Demux1/1
  LPVBlock1/1 -> Radians to Degrees1/1
  Selector/1 -> Sum1/1, Scope14/1, Sum2/2
  Demux1/1 -> Sum3/1, Sum4/2
  Sum2/1 -> Gain4/1
  Sum1/1 -> Gain5/1
  Demux1/2 -> Radians to Degrees/1
  Radians to Degrees/1 -> Scope13/1, Mux8/4
  Gain5/1 -> Scope12/1, Mux8/3
  Gain4/1 -> Scope11/1, Mux8/2
  Radians to Degrees1/1 -> Scope10/1, Mux8/1
  Mux8/1 -> Out/1
  Gain2/1 -> Mux5/4, Scope7/1
  Degrees to Radians1/1 -> Mux5/3
  Degrees to Radians/1 -> Mux5/2
  Mux5/1 -> LPVBlock1/1, Scope/1
  Bus Selector3/1 -> Gain6/1  "<An_c>"
  Bus to Vector1/1 -> Mux5/1
  Bus Selector4/1 -> Bus to Vector/1
  Bus to Vector/1 -> Mux7/1
  Velocity Conversion/1 -> Mux/1
  Demux/2 -> Scope8/1
  Demux/1 -> Scope1/1
  Demux/3 -> Scope9/1
  Gain6/1 -> Scope5/1, Bus to Vector1/1
  Guidance1/1 -> Gain7/1
  Gain7/1 -> Selector/1
  Constant1/1 -> LPVBlock4/1
  [rho] -> LPVBlock4/2
  Sum4/1 -> Sum2/1
  Sum3/1 -> Sum1/2
  Gain8/1 -> Sum4/1, Sum3/2
  LPVBlock4/1 -> Gain8/1
